simulink model "Two_area_LFC"  (R2024a)
settings: Solver=VariableStepAuto  StartTime=0.0  StopTime=50.0  RelTol=1e-3
settings Model: Creator=Sadi  LastModifiedBy=haris
settings SolverCC: AlgebraicLoopSolver=TrustRegion
settings DebuggingCC: UnconnectedInputMsg=warning  UnconnectedOutputMsg=warning  UnconnectedLineMsg=warning
settings ModelReferenceCC: EnableRefExpFcnMdlSchedulingChecks=on
settings RTWCC: GPUComputeCapability=3.5

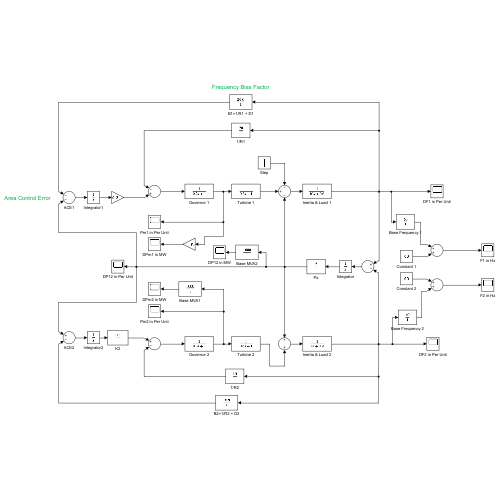
[thumbnail: Simulink's stored preview of the top-level diagram]
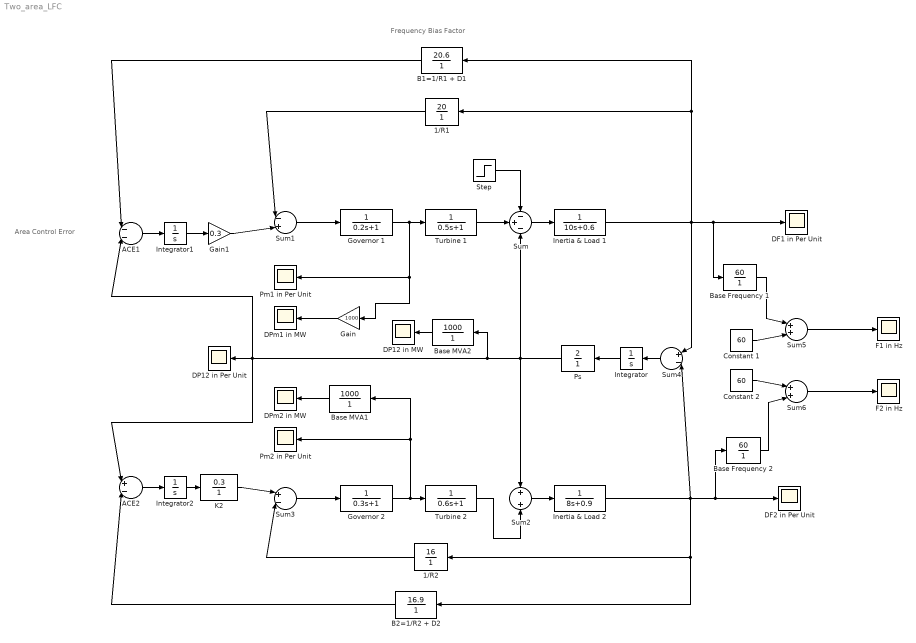
== system Two_area_LFC ==
  note: Area Control Error
  note: Frequency Bias Factor
  1/R1 : TransferFcn  Numerator=[20]  Denominator=[1]
  1/R2 : TransferFcn  Numerator=[16]  Denominator=[1]
  ACE1 : Sum  Inputs=|--|
  ACE2 : Sum  Inputs=|+-|
  B1=1/R1 + D1 : TransferFcn  Numerator=[20.6]  Denominator=[1]
  B2=1/R2 + D2 : TransferFcn  Numerator=[16.9]  Denominator=[1]
  Base Frequency 1 : TransferFcn  Numerator=[60]  Denominator=[1]
  Base Frequency 2 : TransferFcn  Numerator=[60]  Denominator=[1]
  Base MVA1 : TransferFcn  Numerator=[1000]  Denominator=[1]
  Base MVA2 : TransferFcn  Numerator=[1000]  Denominator=[1]
  Constant 1 : Constant  Value=60
  Constant 2 : Constant  Value=60
  DF1 in Per Unit : Scope
  DF2 in Per Unit : Scope
  DP12 in MW : Scope
  DP12 in Per Unit : Scope
  DPm1 in MW : Scope
  DPm2 in MW : Scope
  F1 in Hz : Scope
  F2 in Hz : Scope
  Gain : Gain  Gain=1000
  Gain1 : Gain  Gain=0.3
  Governor 1 : TransferFcn  Denominator=[0.2 1]
  Governor 2 : TransferFcn  Denominator=[0.3 1]
  Inertia & Load 1 : TransferFcn  Denominator=[10 0.6]
  Inertia & Load 2 : TransferFcn  Denominator=[8 0.9]
  Integrator : Integrator
  Integrator1 : Integrator
  Integrator2 : Integrator
  K2 : TransferFcn  Numerator=[0.3]  Denominator=[1]
  Pm1 in Per Unit : Scope
  Pm2 in Per Unit : Scope
  Ps : TransferFcn  Numerator=[2]  Denominator=[1]
  Step : Step  Time=100  Before=0.1875  After=0.1875  SampleTime=0
  Sum : Sum  Inputs=-+-
  Sum1 : Sum  Inputs=|-+|
  Sum2 : Sum
  Sum3 : Sum  Inputs=|+-|
  Sum4 : Sum  Inputs=|+-|
  Sum5 : Sum  Inputs=|++|
  Sum6 : Sum  Inputs=|++|
  Turbine 1 : TransferFcn  Denominator=[0.5 1]
  Turbine 2 : TransferFcn  Denominator=[0.6 1]
  wires:
  Sum1/1 -> Governor 1/1
  Governor 1/1 -> Gain/1, Pm1 in Per Unit/1, Turbine 1/1
  Turbine 1/1 -> Sum/2
  Sum/1 -> Inertia & Load 1/1
  Inertia & Load 1/1 -> B1=1/R1 + D1/1, 1/R1/1, Base Frequency 1/1, DF1 in Per Unit/1, Sum4/1
  1/R1/1 -> Sum1/1
  Turbine 2/1 -> Sum2/2
  Sum3/1 -> Governor 2/1
  Sum2/1 -> Inertia & Load 2/1
  Governor 2/1 -> Base MVA1/1, Pm2 in Per Unit/1, Turbine 2/1
  Sum4/1 -> Integrator/1
  Integrator/1 -> Ps/1
  Ps/1 -> Sum/3, Sum2/1, Base MVA2/1, ACE2/1, ACE1/2, DP12 in Per Unit/1
  Step/1 -> Sum/1
  Base Frequency 1/1 -> Sum5/1
  Base Frequency 2/1 -> Sum6/2
  Inertia & Load 2/1 -> Sum4/2, Base Frequency 2/1, DF2 in Per Unit/1, B2=1/R2 + D2/1, 1/R2/1
  Constant 1/1 -> Sum5/2
  Sum5/1 -> F1 in Hz/1
  Sum6/1 -> F2 in Hz/1
  Constant 2/1 -> Sum6/1
  Gain/1 -> DPm1 in MW/1
  Base MVA1/1 -> DPm2 in MW/1
  ACE1/1 -> Integrator1/1
  B1=1/R1 + D1/1 -> ACE1/1
  Integrator1/1 -> Gain1/1
  Gain1/1 -> Sum1/2
  ACE2/1 -> Integrator2/1
  Integrator2/1 -> K2/1
  B2=1/R2 + D2/1 -> ACE2/2
  1/R2/1 -> Sum3/2
  K2/1 -> Sum3/1
  Base MVA2/1 -> DP12 in MW/1
